simulink model "F1_Simulator"  (R2026a)
settings: Solver=VariableStepAuto  StopTime=260  MaxStep=0.01
values from neighbouring files (symbols this model uses):
  C = [C; C(1,:)]    [f1_corner_map.m]    (also in f1_lateral_tire_table.m = 1.3; f1_sector_map.m = C([true; hypot(diff(C(:,1)), diff(C(:,2))) > 1e-6], :); f1_sensitivity_sweep.m = {; f1_telemetry.m = C([true; hypot(diff(C(:,1)), diff(C(:,2))) > 1e-6], :))
  m = sU >= d0 & sU <= d1    [f1_corner_map.m]    (also in f1_sector_map.m = dC >= edM(k) & dC <= edM(k+1); f1_speed_profile.m = veh.m)
  normalX = -tangentY    [f1_finish_line_params.m]
  normalY = tangentX    [f1_finish_line_params.m]
  s = cumtrapz(tg, v)    [f1_internal_states.m]    (also in f1_track_animation.m = [0; cumsum(hypot(diff(x), diff(y)))]; f1_track_curvature.m = s_all(keepIdx))
  startX = track(1,1)    [f1_finish_line_params.m]
  startY = track(1,2)    [f1_finish_line_params.m]
  tangentX = dirVec(1)    [f1_finish_line_params.m]
  tangentY = dirVec(2)    [f1_finish_line_params.m]
  trackPsi = psi(idx)    [f1_load_raceline.m]    (also in f1_track_curvature.m = atan2(gradient(trackY), gradient(trackX)))
  trackVref = min(trackVref, vf)    [f1_speed_profile.m]
  trackX = x0    [f1_load_raceline.m]    (also in f1_track_curvature.m = x; silverstone_curvature.mat = [-563.032417564 -561.782952087 -560.539483404 -559.300900612)
  trackY = y0    [f1_load_raceline.m]    (also in f1_track_curvature.m = y; silverstone_curvature.mat = [-515.713759288 -514.151171661 -512.584488731 -511.014091481)
undefined symbols (not defined in the file or in its folder): fp_brk_bore, fp_brk_front, fp_brk_maxT, fp_brk_mu_k, fp_brk_pads, fp_brk_Rm, fp_CdA_corner, fp_CdA_straight, fp_eta_tr, fp_gears, fp_h_cg, fp_mu_brake, fp_mu_pk, fp_mu_trac, fp_N_diff, fp_rho, fp_rpm_dn, fp_rpm_lim_end, fp_rpm_lim_ini, fp_rpm_up, fp_track, pwr, veh
libraries: vehdynlibtire x4, autolibsharedcoupling x3, simulink x1, vehdynlibdriver x1, autolibsharedtransfixedgear x1, autolibshareddiff x1, autolibsharedmappedengines x1, autolibshared x1
(part 4 of 5)

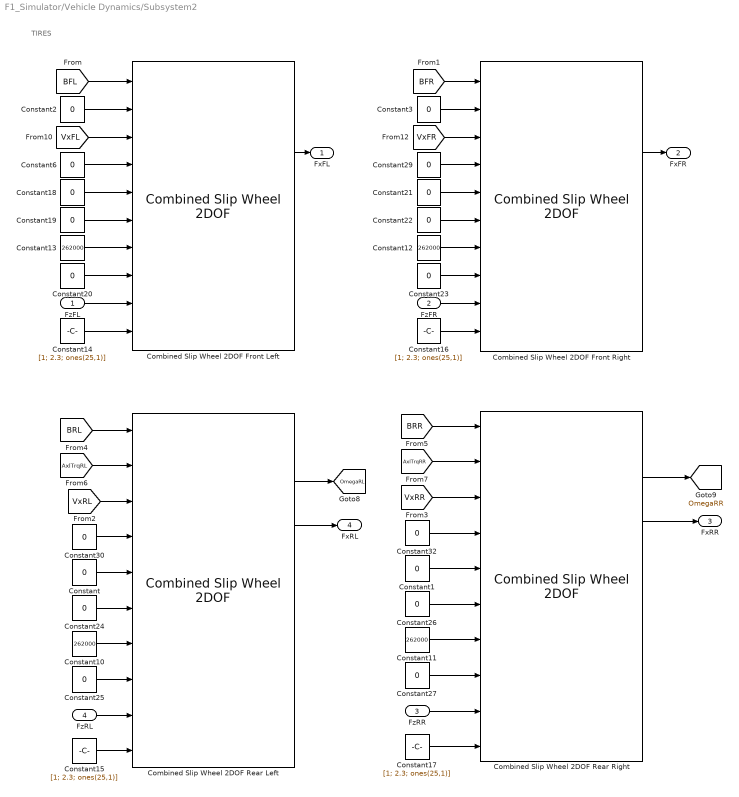
== system F1_Simulator/Vehicle Dynamics/Subsystem2 ==
  note: TIRES
  FzFL : Inport
  FzFR : Inport  Port=2
  FzRR : Inport  Port=3
  FzRL : Inport  Port=4
  Combined Slip Wheel 2DOF Front Left : vehdynlibtire/Combined Slip Wheel 2DOF  tireType=External file  tireParamSet=C:\Users\Julian\Downloads\obfuscated.tir  vertType=Magic Formula  plySteer=on  turnslip=on  BrakeType=Disc  mu_static=0.45  mu_kinetic=brk.mu_k  drum_abore=0.0508  drum_a=0.123  drum_c=0.212  drum_r=0.15  drum_theta1=0  drum_theta2=126  disk_abore=brk.disk_abore  Rm=brk.Rm  num_pads=brk.num_pads  brake_p_bpt=[1 11.4736842105263 21.9473684210526 32.4210526315789 42.8947368421053 53.3684210526316 63.8421052631579 74.3157894736842 84.7894736842105 95.2631578947368 105.736842105263 116.210526315789 126.684210526316 137.157894736842 147.631578947368 158.105263157895 168.578947368421 179.052631578947 189.526315789474 200]  brake_n_bpt=[0 52.6315789473684 105.263157894737 157.894736842105 210.526315789474 263.157894736842 315.789473684211 368.421052631579 421.052631578947 473.684210526316 526.315789473684 578.947368421053 631.578947368421 684.210526315789 736.842105263158 789.473684210526 842.105263157895 894.736842105263 947.368421052632 1000]  f_brake_t=[43.4900602404453 42.5056030554862 41.5350898940194 40.5780454442085 39.6340111501808 38.7025443887544 37.7832176914519 36.8756180088306 35.9793460143796 35.0940154454303 34.2192524787115 33.3546951383474 32.4999927342521 31.6548053290159 30.8188032315107 29.991666515561 29.1730845621415 28.362755623661 27.5603864089927 26.765691687993;498.991217495636 487.695866636631 476.560505099801 465.579679307235 454.748127933653 444.060772460445 433.51270824929 423.099196101319 412.81565427025 402.657650900201 392.620896861006 382.701238955775 372.894653477208 363.197240090814 353.605216024701 344.114910546964 334.722759712992 325.425301366216 316.219170376863 307.10109410434;954.492374750826 932.886130217776 911.585920305583 890.581313170261 869.862244717126 849.419000532136 829.242198807128 809.322774193808 789.651962526121 770.221286354971 751.0225412433 732.047782773203 713.289314220164 694.739674852612 676.391628817892 658.238154578366 640.272434863842 622.48784710877 604.877954344734 587.436496520688;1409.99353200602 1378.07639379892 1346.61133551136 1315.58294703329 1284.9763615006 1254.77722860383 1224.97168936497 1195.5463522863 1166.48827078199 1137.78492180974 1109.42418562559 1081.39432659063 1053.68397496312 1026.28210961441 999.178041611083 972.361398609768 945.822110014692 919.550392851325 893.536738312604 867.771898937035;1865.49468926121 1823.26665738007 1781.63675071715 1740.58458089631 1700.09047828407 1660.13545667552 1620.7011799228 1581.76993037878 1543.32457903786 1505.34855726451 1467.82583000789 1430.74087040806 1394.07863570608 1357.82454437621 1321.96445440427 1286.48464264117 1251.37178516554 1216.61293859388 1182.19552228048 1148.10730135338;2320.9958465164 2268.45692096121 2216.66216592293 2165.58621475934 2115.20459506754 2065.49368474721 2016.43067048064 1967.99350847127 1920.16088729373 1872.91219271928 1826.22747439018 1780.08741422549 1734.47329644903 1689.36697913801 1644.75086719747 1600.60788667257 1556.92146031639 1513.67548433643 1470.85430624835 1428.44270376973;2776.49700377159 2713.64718454235 2651.68758112871 2590.58784862237 2530.31871185102 2470.8519128189 2412.16016103848 2354.21708656376 2296.9971955496 2240.47582817405 2184.62911877248 2129.43395804292 2074.86795719199 2020.9094138998 1967.53727999066 1914.73113070398 1862.47113546724 1810.73803007899 1759.51309021622 1708.77810618608;3231.99816102678 3158.8374481235 3086.71299633449 3015.58948248539 2945.43282863449 2876.21014089059 2807.88965159632 2740.44066465625 2673.83350380547 2608.03946362882 2543.03076315477 2478.78050186034 2415.26261793494 2352.4518486616 2290.32369278385 2228.85437473538 2168.02081061809 2107.80057582154 2048.17187418409 1989.11350860242;3687.49931828197 3604.02771170464 3521.73841154027 3440.59111634842 3360.54694541796 3281.56836896228 3203.61914215416 3126.66424274874 3050.66981206134 2975.60309908359 2901.43240753707 2828.12704567777 2755.6572786779 2683.9942834234 2613.11010557704 2542.97761876678 2473.57048576894 2404.8631215641 2336.83065815196 2269.44891101877;4143.00047553716 4049.21797528579 3956.76382674606 3865.59275021144 3775.66106220143 3686.92659703397 3599.34863271199 3512.88782084123 3427.50612031721 3343.16673453836 3259.83405191936 3177.4735894952 3096.05193942085 3015.5367181852 2935.89651837023 2857.10086279818 2779.12016091979 2701.92566730665 2625.48944211983 2549.78431343512;4598.50163279235 4494.40823886693 4391.78924195184 4290.59438407447 4190.77517898491 4092.28482510566 3995.07812326983 3899.11139893372 3804.34242857308 3710.73036999313 3618.23569630166 3526.82013331263 3436.44660016381 3347.079152947 3258.68293116342 3171.22410682959 3084.66983607064 2998.98821304921 2914.1482260877 2830.11971585147;5054.00279004754 4939.59850244808 4826.81465715762 4715.59601793749 4605.88929576838 4497.64305317735 4390.80761382767 4285.3349770262 4181.17873682896 4078.2940054479 3976.63734068395 3876.16667713006 3776.84126090677 3678.62158770879 3581.46934395661 3485.34735086099 ...(+2764 chars)]  NOMPRES=262000  PRESMAX=1000000  PRESMIN=10000  FNOMIN=tire.Fz0_roll  FZMAX=tire.FZMAX  FZMIN=100  VXLOW=1  KPUMAX=1.5  KPUMIN=-1.5  ALPMAX=1.5  ALPMIN=-1.5  CAMMAX=0.17453  CAMMIN=-0.17453  LONGVL=16.7  FxRelFreqLwrLim=40*pi  FyRelFreqLwrLim=0  MyRelFreqLwrLim=40*pi  omegao=0  UNLOADED_RADIUS=0.353  WIDTH=0.280  RIM_RADIUS=0.2286  ASPECT_RATIO=0.45  MASS=11.2  IYY=1.084  br=0.01  GRAVITY=-9.81  zo=0  zdoto=0  BREFF=8.25094594147963  DREFF=0.260468730454265  FREFF=0.0735298544471851  Q_RE0=1.00866439868088  Q_V1=0.000760413786224011  Q_V2=0.0463384792019201  Q_FZ1=0  Q_FZ2=15.6870832810226  Q_FZ3=0  Q_FCX=0.138643970247602  Q_FCY=0.10843499565426  Q_FCY2=-0.465763352339538  PFZ1=0.69958166705601  VERTICAL_STIFFNESS=207885.061134007  VERTICAL_DAMPING=500  BOTTOM_OFFST=0.00990653336182505  BOTTOM_STIFF=1999075.87051971  Q_CAM1=86.7791723017291  Q_CAM2=259.705254231766  Q_CAM3=0.510281667378416  Q_FYS1=-20769.4728880343  Q_FYS2=-59060.183485617  Q_FYS3=89271.8260126986  LONGITUDINAL_STIFFNESS=388714.175879854  LATERAL_STIFFNESS=157087.404633332  PCFX1=0.18539229191199  PCFX2=0  PCFX3=0  PCFY1=0.163183345037677  PCFY2=0  PCFY3=0.249094918231954  Q_RA1=0.675942571700787  Q_RA2=0.73800463546164  Q_RB1=1.04487486456705  Q_RB2=-1.191763806629  PCX1=1.58523057950359  PDX1=1.7  PDX2=-0.0842405110022724  PDX3=0  PEX1=0.110312777158455  PEX2=0.313468516038146  PEX3=0  PEX4=0.0016060905760045  PKX1=21.3872544684023  PKX2=14.0006541873175  PKX3=-0.405326109653452  PHX1=0.000212599305364818  PHX2=0.00115950515263055  PVX1=1.59236164471432e-05  PVX2=0.000104321112127671  PPX1=-0.349461321276586  PPX2=0.387840040616429  PPX3=-0.0969947336569324  PPX4=0.0632271859795801  RBX1=12.7633329850276  RBX2=9.5787123658471  RBX3=0  RCX1=1.02796280922059  REX1=-0.45202516851367  REX2=-0.47304886171176  RHX1=0.000233272373115809  QSX1=-0.00788307788961443  QSX2=0.954629515459396  QSX3=0.0155855777667025  QSX4=0.125904607142414  QSX5=1.01110069703963  QSX6=20.1938577118433  QSX7=0.310818120717083  QSX8=-0.0430823751139655  QSX9=0.636494404888216  QSX10=0.142438060591663  QSX11=0.346766530036373  QSX12=0  QSX13=0  QSX14=0  PPMX1=0  PCY1=1.34299950037631  PDY1=0.878267729082195  PDY2=-0.0644597923147385  PDY3=0  PEY1=-0.809776534470972  PEY2=-0.600180598867198  PEY3=0.0991732552633487  PEY4=-6.5577974035573  PEY5=0  PKY1=-15.5714726518315  PKY2=1.73126522291751  PKY3=0.365349873517229  PKY4=1.98176755955416  PKY5=0  PKY6=-0.884005199550313  PKY7=-0.237259727611847  PHY1=-0.00183370557235628  PHY2=0.00346401302716671  PVY1=-0.00675427560163264  PVY2=0.036379218103843  PVY3=-0.163543984089166  PVY4=-0.491003349625726  PPY1=-0.62059646553185  PPY2=-0.0647824842338686  PPY3=-0.164648843290686  PPY4=0.283193909060098  PPY5=0  RBY1=10.7588809173639  RBY2=7.70420065295029  RBY3=3.40283755070691e-06  RBY4=0  RCY1=1.06691874059059  REY1=0.308244924574305  REY2=7.48775032604508e-06  RHY1=0.0118479204960415  RHY2=7.63650177161071e-06  RVY1=0.0560024425050078  RVY2=7.48487127056197e-06  RVY3=0  RVY4=98.4047026517149  RVY5=2.02759273900054  RVY6=15.7623064923347  QSY1=0.00699077564863536  QSY2=0  QSY3=0.00153535478298811  QSY4=8.55710322455322e-05  QSY5=0  QSY6=0  QSY7=0.89443879773793  QSY8=-0.403227641260894  QBZ1=11.666656027484  QBZ2=-1.30355438574485  QBZ3=0  QBZ4=0.177918305399071  QBZ5=-0.162481135068033  QBZ6=0  QBZ9=30.1445534682089  QBZ10=0  QCZ1=1.29026978207574  QDZ1=0.0886972644991399  QDZ2=-0.0058634820161856  QDZ3=0.3805597481383  QDZ4=0  QDZ6=0.00160914918118959  QDZ7=-0.00211036330862154  QDZ8=-0.13921904912557  QDZ9=0.00816585550028243  QDZ10=0  QDZ11=0  QEZ1=-2.19802254534746  QEZ2=1.01850535789165  QEZ3=0  QEZ4=0.278379679112054  QEZ5=-0.548414722765386  QHZ1=0.00148361198869669  QHZ2=0.00202017567585904  QHZ3=0.240316641332066  QHZ4=-0.210114035738085  PPZ1=-0.443927982388615  PPZ2=0  SSZ1=0.00914999585397887  SSZ2=0.0389830656052735  SSZ3=0  SSZ4=0  PDXP1=0.396718274678791  PDXP2=0  PDXP3=0  PKYP1=1.00587060633573  PDYP1=0.40483048923438  PDYP2=0  PDYP3=0  PDYP4=0  PHYP1=0.992731942067188  PHYP2=0.150352945499914  PHYP3=0  PHYP4=-3.98988682633674  PECP1=0.502379254513503  PECP2=0  QDTP1=10.0178654287947  QCRP1=0.200627747200702  QCRP2=0.0995735881599772  QBRP1=0.0997107127960717  QDRP1=1.01432910167423  QDRP2=0  aMode=2
  Combined Slip Wheel 2DOF Front Right : vehdynlibtire/Combined Slip Wheel 2DOF  tireType=External file  tireParamSet=C:\Users\Julian\Downloads\obfuscated.tir  vertType=Magic Formula  plySteer=on  turnslip=on  BrakeType=Disc  mu_static=0.45  mu_kinetic=brk.mu_k  drum_abore=0.0508  drum_a=0.123  drum_c=0.212  drum_r=0.15  drum_theta1=0  drum_theta2=126  disk_abore=brk.disk_abore  Rm=brk.Rm  num_pads=brk.num_pads  brake_p_bpt=[1 11.4736842105263 21.9473684210526 32.4210526315789 42.8947368421053 53.3684210526316 63.8421052631579 74.3157894736842 84.7894736842105 95.2631578947368 105.736842105263 116.210526315789 126.684210526316 137.157894736842 147.631578947368 158.105263157895 168.578947368421 179.052631578947 189.526315789474 200]  brake_n_bpt=[0 52.6315789473684 105.263157894737 157.894736842105 210.526315789474 263.157894736842 315.789473684211 368.421052631579 421.052631578947 473.684210526316 526.315789473684 578.947368421053 631.578947368421 684.210526315789 736.842105263158 789.473684210526 842.105263157895 894.736842105263 947.368421052632 1000]  f_brake_t=[43.4900602404453 42.5056030554862 41.5350898940194 40.5780454442085 39.6340111501808 38.7025443887544 37.7832176914519 36.8756180088306 35.9793460143796 35.0940154454303 34.2192524787115 33.3546951383474 32.4999927342521 31.6548053290159 30.8188032315107 29.991666515561 29.1730845621415 28.362755623661 27.5603864089927 26.765691687993;498.991217495636 487.695866636631 476.560505099801 465.579679307235 454.748127933653 444.060772460445 433.51270824929 423.099196101319 412.81565427025 402.657650900201 392.620896861006 382.701238955775 372.894653477208 363.197240090814 353.605216024701 344.114910546964 334.722759712992 325.425301366216 316.219170376863 307.10109410434;954.492374750826 932.886130217776 911.585920305583 890.581313170261 869.862244717126 849.419000532136 829.242198807128 809.322774193808 789.651962526121 770.221286354971 751.0225412433 732.047782773203 713.289314220164 694.739674852612 676.391628817892 658.238154578366 640.272434863842 622.48784710877 604.877954344734 587.436496520688;1409.99353200602 1378.07639379892 1346.61133551136 1315.58294703329 1284.9763615006 1254.77722860383 1224.97168936497 1195.5463522863 1166.48827078199 1137.78492180974 1109.42418562559 1081.39432659063 1053.68397496312 1026.28210961441 999.178041611083 972.361398609768 945.822110014692 919.550392851325 893.536738312604 867.771898937035;1865.49468926121 1823.26665738007 1781.63675071715 1740.58458089631 1700.09047828407 1660.13545667552 1620.7011799228 1581.76993037878 1543.32457903786 1505.34855726451 1467.82583000789 1430.74087040806 1394.07863570608 1357.82454437621 1321.96445440427 1286.48464264117 1251.37178516554 1216.61293859388 1182.19552228048 1148.10730135338;2320.9958465164 2268.45692096121 2216.66216592293 2165.58621475934 2115.20459506754 2065.49368474721 2016.43067048064 1967.99350847127 1920.16088729373 1872.91219271928 1826.22747439018 1780.08741422549 1734.47329644903 1689.36697913801 1644.75086719747 1600.60788667257 1556.92146031639 1513.67548433643 1470.85430624835 1428.44270376973;2776.49700377159 2713.64718454235 2651.68758112871 2590.58784862237 2530.31871185102 2470.8519128189 2412.16016103848 2354.21708656376 2296.9971955496 2240.47582817405 2184.62911877248 2129.43395804292 2074.86795719199 2020.9094138998 1967.53727999066 1914.73113070398 1862.47113546724 1810.73803007899 1759.51309021622 1708.77810618608;3231.99816102678 3158.8374481235 3086.71299633449 3015.58948248539 2945.43282863449 2876.21014089059 2807.88965159632 2740.44066465625 2673.83350380547 2608.03946362882 2543.03076315477 2478.78050186034 2415.26261793494 2352.4518486616 2290.32369278385 2228.85437473538 2168.02081061809 2107.80057582154 2048.17187418409 1989.11350860242;3687.49931828197 3604.02771170464 3521.73841154027 3440.59111634842 3360.54694541796 3281.56836896228 3203.61914215416 3126.66424274874 3050.66981206134 2975.60309908359 2901.43240753707 2828.12704567777 2755.6572786779 2683.9942834234 2613.11010557704 2542.97761876678 2473.57048576894 2404.8631215641 2336.83065815196 2269.44891101877;4143.00047553716 4049.21797528579 3956.76382674606 3865.59275021144 3775.66106220143 3686.92659703397 3599.34863271199 3512.88782084123 3427.50612031721 3343.16673453836 3259.83405191936 3177.4735894952 3096.05193942085 3015.5367181852 2935.89651837023 2857.10086279818 2779.12016091979 2701.92566730665 2625.48944211983 2549.78431343512;4598.50163279235 4494.40823886693 4391.78924195184 4290.59438407447 4190.77517898491 4092.28482510566 3995.07812326983 3899.11139893372 3804.34242857308 3710.73036999313 3618.23569630166 3526.82013331263 3436.44660016381 3347.079152947 3258.68293116342 3171.22410682959 3084.66983607064 2998.98821304921 2914.1482260877 2830.11971585147;5054.00279004754 4939.59850244808 4826.81465715762 4715.59601793749 4605.88929576838 4497.64305317735 4390.80761382767 4285.3349770262 4181.17873682896 4078.2940054479 3976.63734068395 3876.16667713006 3776.84126090677 3678.62158770879 3581.46934395661 3485.34735086099 ...(+2764 chars)]  NOMPRES=262000  PRESMAX=1000000  PRESMIN=10000  FNOMIN=tire.Fz0_roll  FZMAX=tire.FZMAX  FZMIN=100  VXLOW=1  KPUMAX=1.5  KPUMIN=-1.5  ALPMAX=1.5  ALPMIN=-1.5  CAMMAX=0.17453  CAMMIN=-0.17453  LONGVL=16.7  FxRelFreqLwrLim=40*pi  FyRelFreqLwrLim=0  MyRelFreqLwrLim=40*pi  omegao=0  UNLOADED_RADIUS=0.353  WIDTH=0.280  RIM_RADIUS=0.2286  ASPECT_RATIO=0.45  MASS=11.2  IYY=1.084  br=0.01  GRAVITY=-9.81  zo=0  zdoto=0  BREFF=8.25094594147963  DREFF=0.260468730454265  FREFF=0.0735298544471851  Q_RE0=1.00866439868088  Q_V1=0.000760413786224011  Q_V2=0.0463384792019201  Q_FZ1=0  Q_FZ2=15.6870832810226  Q_FZ3=0  Q_FCX=0.138643970247602  Q_FCY=0.10843499565426  Q_FCY2=-0.465763352339538  PFZ1=0.69958166705601  VERTICAL_STIFFNESS=207885.061134007  VERTICAL_DAMPING=500  BOTTOM_OFFST=0.00990653336182505  BOTTOM_STIFF=1999075.87051971  Q_CAM1=86.7791723017291  Q_CAM2=259.705254231766  Q_CAM3=0.510281667378416  Q_FYS1=-20769.4728880343  Q_FYS2=-59060.183485617  Q_FYS3=89271.8260126986  LONGITUDINAL_STIFFNESS=388714.175879854  LATERAL_STIFFNESS=157087.404633332  PCFX1=0.18539229191199  PCFX2=0  PCFX3=0  PCFY1=0.163183345037677  PCFY2=0  PCFY3=0.249094918231954  Q_RA1=0.675942571700787  Q_RA2=0.73800463546164  Q_RB1=1.04487486456705  Q_RB2=-1.191763806629  PCX1=1.58523057950359  PDX1=1.7  PDX2=-0.0842405110022724  PDX3=0  PEX1=0.110312777158455  PEX2=0.313468516038146  PEX3=0  PEX4=0.0016060905760045  PKX1=21.3872544684023  PKX2=14.0006541873175  PKX3=-0.405326109653452  PHX1=0.000212599305364818  PHX2=0.00115950515263055  PVX1=1.59236164471432e-05  PVX2=0.000104321112127671  PPX1=-0.349461321276586  PPX2=0.387840040616429  PPX3=-0.0969947336569324  PPX4=0.0632271859795801  RBX1=12.7633329850276  RBX2=9.5787123658471  RBX3=0  RCX1=1.02796280922059  REX1=-0.45202516851367  REX2=-0.47304886171176  RHX1=0.000233272373115809  QSX1=-0.00788307788961443  QSX2=0.954629515459396  QSX3=0.0155855777667025  QSX4=0.125904607142414  QSX5=1.01110069703963  QSX6=20.1938577118433  QSX7=0.310818120717083  QSX8=-0.0430823751139655  QSX9=0.636494404888216  QSX10=0.142438060591663  QSX11=0.346766530036373  QSX12=0  QSX13=0  QSX14=0  PPMX1=0  PCY1=1.34299950037631  PDY1=0.878267729082195  PDY2=-0.0644597923147385  PDY3=0  PEY1=-0.809776534470972  PEY2=-0.600180598867198  PEY3=0.0991732552633487  PEY4=-6.5577974035573  PEY5=0  PKY1=-15.5714726518315  PKY2=1.73126522291751  PKY3=0.365349873517229  PKY4=1.98176755955416  PKY5=0  PKY6=-0.884005199550313  PKY7=-0.237259727611847  PHY1=-0.00183370557235628  PHY2=0.00346401302716671  PVY1=-0.00675427560163264  PVY2=0.036379218103843  PVY3=-0.163543984089166  PVY4=-0.491003349625726  PPY1=-0.62059646553185  PPY2=-0.0647824842338686  PPY3=-0.164648843290686  PPY4=0.283193909060098  PPY5=0  RBY1=10.7588809173639  RBY2=7.70420065295029  RBY3=3.40283755070691e-06  RBY4=0  RCY1=1.06691874059059  REY1=0.308244924574305  REY2=7.48775032604508e-06  RHY1=0.0118479204960415  RHY2=7.63650177161071e-06  RVY1=0.0560024425050078  RVY2=7.48487127056197e-06  RVY3=0  RVY4=98.4047026517149  RVY5=2.02759273900054  RVY6=15.7623064923347  QSY1=0.00699077564863536  QSY2=0  QSY3=0.00153535478298811  QSY4=8.55710322455322e-05  QSY5=0  QSY6=0  QSY7=0.89443879773793  QSY8=-0.403227641260894  QBZ1=11.666656027484  QBZ2=-1.30355438574485  QBZ3=0  QBZ4=0.177918305399071  QBZ5=-0.162481135068033  QBZ6=0  QBZ9=30.1445534682089  QBZ10=0  QCZ1=1.29026978207574  QDZ1=0.0886972644991399  QDZ2=-0.0058634820161856  QDZ3=0.3805597481383  QDZ4=0  QDZ6=0.00160914918118959  QDZ7=-0.00211036330862154  QDZ8=-0.13921904912557  QDZ9=0.00816585550028243  QDZ10=0  QDZ11=0  QEZ1=-2.19802254534746  QEZ2=1.01850535789165  QEZ3=0  QEZ4=0.278379679112054  QEZ5=-0.548414722765386  QHZ1=0.00148361198869669  QHZ2=0.00202017567585904  QHZ3=0.240316641332066  QHZ4=-0.210114035738085  PPZ1=-0.443927982388615  PPZ2=0  SSZ1=0.00914999585397887  SSZ2=0.0389830656052735  SSZ3=0  SSZ4=0  PDXP1=0.396718274678791  PDXP2=0  PDXP3=0  PKYP1=1.00587060633573  PDYP1=0.40483048923438  PDYP2=0  PDYP3=0  PDYP4=0  PHYP1=0.992731942067188  PHYP2=0.150352945499914  PHYP3=0  PHYP4=-3.98988682633674  PECP1=0.502379254513503  PECP2=0  QDTP1=10.0178654287947  QCRP1=0.200627747200702  QCRP2=0.0995735881599772  QBRP1=0.0997107127960717  QDRP1=1.01432910167423  QDRP2=0  aMode=2
  Combined Slip Wheel 2DOF Rear Left : vehdynlibtire/Combined Slip Wheel 2DOF  tireType=External file  tireParamSet=C:\Users\Julian\Downloads\obfuscated.tir  vertType=Magic Formula  plySteer=on  turnslip=on  BrakeType=Disc  mu_static=0.45  mu_kinetic=brk.mu_k  drum_abore=0.0508  drum_a=0.123  drum_c=0.212  drum_r=0.15  drum_theta1=0  drum_theta2=126  disk_abore=brk.disk_abore  Rm=brk.Rm  num_pads=brk.num_pads  brake_p_bpt=[1 11.4736842105263 21.9473684210526 32.4210526315789 42.8947368421053 53.3684210526316 63.8421052631579 74.3157894736842 84.7894736842105 95.2631578947368 105.736842105263 116.210526315789 126.684210526316 137.157894736842 147.631578947368 158.105263157895 168.578947368421 179.052631578947 189.526315789474 200]  brake_n_bpt=[0 52.6315789473684 105.263157894737 157.894736842105 210.526315789474 263.157894736842 315.789473684211 368.421052631579 421.052631578947 473.684210526316 526.315789473684 578.947368421053 631.578947368421 684.210526315789 736.842105263158 789.473684210526 842.105263157895 894.736842105263 947.368421052632 1000]  f_brake_t=[43.4900602404453 42.5056030554862 41.5350898940194 40.5780454442085 39.6340111501808 38.7025443887544 37.7832176914519 36.8756180088306 35.9793460143796 35.0940154454303 34.2192524787115 33.3546951383474 32.4999927342521 31.6548053290159 30.8188032315107 29.991666515561 29.1730845621415 28.362755623661 27.5603864089927 26.765691687993;498.991217495636 487.695866636631 476.560505099801 465.579679307235 454.748127933653 444.060772460445 433.51270824929 423.099196101319 412.81565427025 402.657650900201 392.620896861006 382.701238955775 372.894653477208 363.197240090814 353.605216024701 344.114910546964 334.722759712992 325.425301366216 316.219170376863 307.10109410434;954.492374750826 932.886130217776 911.585920305583 890.581313170261 869.862244717126 849.419000532136 829.242198807128 809.322774193808 789.651962526121 770.221286354971 751.0225412433 732.047782773203 713.289314220164 694.739674852612 676.391628817892 658.238154578366 640.272434863842 622.48784710877 604.877954344734 587.436496520688;1409.99353200602 1378.07639379892 1346.61133551136 1315.58294703329 1284.9763615006 1254.77722860383 1224.97168936497 1195.5463522863 1166.48827078199 1137.78492180974 1109.42418562559 1081.39432659063 1053.68397496312 1026.28210961441 999.178041611083 972.361398609768 945.822110014692 919.550392851325 893.536738312604 867.771898937035;1865.49468926121 1823.26665738007 1781.63675071715 1740.58458089631 1700.09047828407 1660.13545667552 1620.7011799228 1581.76993037878 1543.32457903786 1505.34855726451 1467.82583000789 1430.74087040806 1394.07863570608 1357.82454437621 1321.96445440427 1286.48464264117 1251.37178516554 1216.61293859388 1182.19552228048 1148.10730135338;2320.9958465164 2268.45692096121 2216.66216592293 2165.58621475934 2115.20459506754 2065.49368474721 2016.43067048064 1967.99350847127 1920.16088729373 1872.91219271928 1826.22747439018 1780.08741422549 1734.47329644903 1689.36697913801 1644.75086719747 1600.60788667257 1556.92146031639 1513.67548433643 1470.85430624835 1428.44270376973;2776.49700377159 2713.64718454235 2651.68758112871 2590.58784862237 2530.31871185102 2470.8519128189 2412.16016103848 2354.21708656376 2296.9971955496 2240.47582817405 2184.62911877248 2129.43395804292 2074.86795719199 2020.9094138998 1967.53727999066 1914.73113070398 1862.47113546724 1810.73803007899 1759.51309021622 1708.77810618608;3231.99816102678 3158.8374481235 3086.71299633449 3015.58948248539 2945.43282863449 2876.21014089059 2807.88965159632 2740.44066465625 2673.83350380547 2608.03946362882 2543.03076315477 2478.78050186034 2415.26261793494 2352.4518486616 2290.32369278385 2228.85437473538 2168.02081061809 2107.80057582154 2048.17187418409 1989.11350860242;3687.49931828197 3604.02771170464 3521.73841154027 3440.59111634842 3360.54694541796 3281.56836896228 3203.61914215416 3126.66424274874 3050.66981206134 2975.60309908359 2901.43240753707 2828.12704567777 2755.6572786779 2683.9942834234 2613.11010557704 2542.97761876678 2473.57048576894 2404.8631215641 2336.83065815196 2269.44891101877;4143.00047553716 4049.21797528579 3956.76382674606 3865.59275021144 3775.66106220143 3686.92659703397 3599.34863271199 3512.88782084123 3427.50612031721 3343.16673453836 3259.83405191936 3177.4735894952 3096.05193942085 3015.5367181852 2935.89651837023 2857.10086279818 2779.12016091979 2701.92566730665 2625.48944211983 2549.78431343512;4598.50163279235 4494.40823886693 4391.78924195184 4290.59438407447 4190.77517898491 4092.28482510566 3995.07812326983 3899.11139893372 3804.34242857308 3710.73036999313 3618.23569630166 3526.82013331263 3436.44660016381 3347.079152947 3258.68293116342 3171.22410682959 3084.66983607064 2998.98821304921 2914.1482260877 2830.11971585147;5054.00279004754 4939.59850244808 4826.81465715762 4715.59601793749 4605.88929576838 4497.64305317735 4390.80761382767 4285.3349770262 4181.17873682896 4078.2940054479 3976.63734068395 3876.16667713006 3776.84126090677 3678.62158770879 3581.46934395661 3485.34735086099 ...(+2764 chars)]  NOMPRES=262000  PRESMAX=1000000  PRESMIN=10000  FNOMIN=tire.Fz0_roll  FZMAX=tire.FZMAX  FZMIN=100  VXLOW=1  KPUMAX=1.5  KPUMIN=-1.5  ALPMAX=1.5  ALPMIN=-1.5  CAMMAX=0.17453  CAMMIN=-0.17453  LONGVL=16.7  FxRelFreqLwrLim=40*pi  FyRelFreqLwrLim=0  MyRelFreqLwrLim=40*pi  omegao=0  UNLOADED_RADIUS=0.353  WIDTH=0.375  RIM_RADIUS=0.2286  ASPECT_RATIO=0.45  MASS=11.2  IYY=1.084  br=0.01  GRAVITY=-9.81  zo=0  zdoto=0  BREFF=8.25094594147963  DREFF=0.260468730454265  FREFF=0.0735298544471851  Q_RE0=1.00866439868088  Q_V1=0.000760413786224011  Q_V2=0.0463384792019201  Q_FZ1=0  Q_FZ2=15.6870832810226  Q_FZ3=0  Q_FCX=0.138643970247602  Q_FCY=0.10843499565426  Q_FCY2=-0.465763352339538  PFZ1=0.69958166705601  VERTICAL_STIFFNESS=207885.061134007  VERTICAL_DAMPING=500  BOTTOM_OFFST=0.00990653336182505  BOTTOM_STIFF=1999075.87051971  Q_CAM1=86.7791723017291  Q_CAM2=259.705254231766  Q_CAM3=0.510281667378416  Q_FYS1=-20769.4728880343  Q_FYS2=-59060.183485617  Q_FYS3=89271.8260126986  LONGITUDINAL_STIFFNESS=388714.175879854  LATERAL_STIFFNESS=157087.404633332  PCFX1=0.18539229191199  PCFX2=0  PCFX3=0  PCFY1=0.163183345037677  PCFY2=0  PCFY3=0.249094918231954  Q_RA1=0.675942571700787  Q_RA2=0.73800463546164  Q_RB1=1.04487486456705  Q_RB2=-1.191763806629  PCX1=1.58523057950359  PDX1=1.7  PDX2=-0.0842405110022724  PDX3=0  PEX1=0.110312777158455  PEX2=0.313468516038146  PEX3=0  PEX4=0.0016060905760045  PKX1=21.3872544684023  PKX2=14.0006541873175  PKX3=-0.405326109653452  PHX1=0.000212599305364818  PHX2=0.00115950515263055  PVX1=1.59236164471432e-05  PVX2=0.000104321112127671  PPX1=-0.349461321276586  PPX2=0.387840040616429  PPX3=-0.0969947336569324  PPX4=0.0632271859795801  RBX1=12.7633329850276  RBX2=9.5787123658471  RBX3=0  RCX1=1.02796280922059  REX1=-0.45202516851367  REX2=-0.47304886171176  RHX1=0.000233272373115809  QSX1=-0.00788307788961443  QSX2=0.954629515459396  QSX3=0.0155855777667025  QSX4=0.125904607142414  QSX5=1.01110069703963  QSX6=20.1938577118433  QSX7=0.310818120717083  QSX8=-0.0430823751139655  QSX9=0.636494404888216  QSX10=0.142438060591663  QSX11=0.346766530036373  QSX12=0  QSX13=0  QSX14=0  PPMX1=0  PCY1=1.34299950037631  PDY1=0.878267729082195  PDY2=-0.0644597923147385  PDY3=0  PEY1=-0.809776534470972  PEY2=-0.600180598867198  PEY3=0.0991732552633487  PEY4=-6.5577974035573  PEY5=0  PKY1=-15.5714726518315  PKY2=1.73126522291751  PKY3=0.365349873517229  PKY4=1.98176755955416  PKY5=0  PKY6=-0.884005199550313  PKY7=-0.237259727611847  PHY1=-0.00183370557235628  PHY2=0.00346401302716671  PVY1=-0.00675427560163264  PVY2=0.036379218103843  PVY3=-0.163543984089166  PVY4=-0.491003349625726  PPY1=-0.62059646553185  PPY2=-0.0647824842338686  PPY3=-0.164648843290686  PPY4=0.283193909060098  PPY5=0  RBY1=10.7588809173639  RBY2=7.70420065295029  RBY3=3.40283755070691e-06  RBY4=0  RCY1=1.06691874059059  REY1=0.308244924574305  REY2=7.48775032604508e-06  RHY1=0.0118479204960415  RHY2=7.63650177161071e-06  RVY1=0.0560024425050078  RVY2=7.48487127056197e-06  RVY3=0  RVY4=98.4047026517149  RVY5=2.02759273900054  RVY6=15.7623064923347  QSY1=0.00699077564863536  QSY2=0  QSY3=0.00153535478298811  QSY4=8.55710322455322e-05  QSY5=0  QSY6=0  QSY7=0.89443879773793  QSY8=-0.403227641260894  QBZ1=11.666656027484  QBZ2=-1.30355438574485  QBZ3=0  QBZ4=0.177918305399071  QBZ5=-0.162481135068033  QBZ6=0  QBZ9=30.1445534682089  QBZ10=0  QCZ1=1.29026978207574  QDZ1=0.0886972644991399  QDZ2=-0.0058634820161856  QDZ3=0.3805597481383  QDZ4=0  QDZ6=0.00160914918118959  QDZ7=-0.00211036330862154  QDZ8=-0.13921904912557  QDZ9=0.00816585550028243  QDZ10=0  QDZ11=0  QEZ1=-2.19802254534746  QEZ2=1.01850535789165  QEZ3=0  QEZ4=0.278379679112054  QEZ5=-0.548414722765386  QHZ1=0.00148361198869669  QHZ2=0.00202017567585904  QHZ3=0.240316641332066  QHZ4=-0.210114035738085  PPZ1=-0.443927982388615  PPZ2=0  SSZ1=0.00914999585397887  SSZ2=0.0389830656052735  SSZ3=0  SSZ4=0  PDXP1=0.396718274678791  PDXP2=0  PDXP3=0  PKYP1=1.00587060633573  PDYP1=0.40483048923438  PDYP2=0  PDYP3=0  PDYP4=0  PHYP1=0.992731942067188  PHYP2=0.150352945499914  PHYP3=0  PHYP4=-3.98988682633674  PECP1=0.502379254513503  PECP2=0  QDTP1=10.0178654287947  QCRP1=0.200627747200702  QCRP2=0.0995735881599772  QBRP1=0.0997107127960717  QDRP1=1.01432910167423  QDRP2=0  aMode=2
  Combined Slip Wheel 2DOF Rear Right : vehdynlibtire/Combined Slip Wheel 2DOF  tireType=External file  tireParamSet=C:\Users\Julian\Downloads\obfuscated.tir  vertType=Magic Formula  plySteer=on  turnslip=on  BrakeType=Disc  mu_static=0.45  mu_kinetic=brk.mu_k  drum_abore=0.0508  drum_a=0.123  drum_c=0.212  drum_r=0.15  drum_theta1=0  drum_theta2=126  disk_abore=brk.disk_abore  Rm=brk.Rm  num_pads=brk.num_pads  brake_p_bpt=[1 11.4736842105263 21.9473684210526 32.4210526315789 42.8947368421053 53.3684210526316 63.8421052631579 74.3157894736842 84.7894736842105 95.2631578947368 105.736842105263 116.210526315789 126.684210526316 137.157894736842 147.631578947368 158.105263157895 168.578947368421 179.052631578947 189.526315789474 200]  brake_n_bpt=[0 52.6315789473684 105.263157894737 157.894736842105 210.526315789474 263.157894736842 315.789473684211 368.421052631579 421.052631578947 473.684210526316 526.315789473684 578.947368421053 631.578947368421 684.210526315789 736.842105263158 789.473684210526 842.105263157895 894.736842105263 947.368421052632 1000]  f_brake_t=[43.4900602404453 42.5056030554862 41.5350898940194 40.5780454442085 39.6340111501808 38.7025443887544 37.7832176914519 36.8756180088306 35.9793460143796 35.0940154454303 34.2192524787115 33.3546951383474 32.4999927342521 31.6548053290159 30.8188032315107 29.991666515561 29.1730845621415 28.362755623661 27.5603864089927 26.765691687993;498.991217495636 487.695866636631 476.560505099801 465.579679307235 454.748127933653 444.060772460445 433.51270824929 423.099196101319 412.81565427025 402.657650900201 392.620896861006 382.701238955775 372.894653477208 363.197240090814 353.605216024701 344.114910546964 334.722759712992 325.425301366216 316.219170376863 307.10109410434;954.492374750826 932.886130217776 911.585920305583 890.581313170261 869.862244717126 849.419000532136 829.242198807128 809.322774193808 789.651962526121 770.221286354971 751.0225412433 732.047782773203 713.289314220164 694.739674852612 676.391628817892 658.238154578366 640.272434863842 622.48784710877 604.877954344734 587.436496520688;1409.99353200602 1378.07639379892 1346.61133551136 1315.58294703329 1284.9763615006 1254.77722860383 1224.97168936497 1195.5463522863 1166.48827078199 1137.78492180974 1109.42418562559 1081.39432659063 1053.68397496312 1026.28210961441 999.178041611083 972.361398609768 945.822110014692 919.550392851325 893.536738312604 867.771898937035;1865.49468926121 1823.26665738007 1781.63675071715 1740.58458089631 1700.09047828407 1660.13545667552 1620.7011799228 1581.76993037878 1543.32457903786 1505.34855726451 1467.82583000789 1430.74087040806 1394.07863570608 1357.82454437621 1321.96445440427 1286.48464264117 1251.37178516554 1216.61293859388 1182.19552228048 1148.10730135338;2320.9958465164 2268.45692096121 2216.66216592293 2165.58621475934 2115.20459506754 2065.49368474721 2016.43067048064 1967.99350847127 1920.16088729373 1872.91219271928 1826.22747439018 1780.08741422549 1734.47329644903 1689.36697913801 1644.75086719747 1600.60788667257 1556.92146031639 1513.67548433643 1470.85430624835 1428.44270376973;2776.49700377159 2713.64718454235 2651.68758112871 2590.58784862237 2530.31871185102 2470.8519128189 2412.16016103848 2354.21708656376 2296.9971955496 2240.47582817405 2184.62911877248 2129.43395804292 2074.86795719199 2020.9094138998 1967.53727999066 1914.73113070398 1862.47113546724 1810.73803007899 1759.51309021622 1708.77810618608;3231.99816102678 3158.8374481235 3086.71299633449 3015.58948248539 2945.43282863449 2876.21014089059 2807.88965159632 2740.44066465625 2673.83350380547 2608.03946362882 2543.03076315477 2478.78050186034 2415.26261793494 2352.4518486616 2290.32369278385 2228.85437473538 2168.02081061809 2107.80057582154 2048.17187418409 1989.11350860242;3687.49931828197 3604.02771170464 3521.73841154027 3440.59111634842 3360.54694541796 3281.56836896228 3203.61914215416 3126.66424274874 3050.66981206134 2975.60309908359 2901.43240753707 2828.12704567777 2755.6572786779 2683.9942834234 2613.11010557704 2542.97761876678 2473.57048576894 2404.8631215641 2336.83065815196 2269.44891101877;4143.00047553716 4049.21797528579 3956.76382674606 3865.59275021144 3775.66106220143 3686.92659703397 3599.34863271199 3512.88782084123 3427.50612031721 3343.16673453836 3259.83405191936 3177.4735894952 3096.05193942085 3015.5367181852 2935.89651837023 2857.10086279818 2779.12016091979 2701.92566730665 2625.48944211983 2549.78431343512;4598.50163279235 4494.40823886693 4391.78924195184 4290.59438407447 4190.77517898491 4092.28482510566 3995.07812326983 3899.11139893372 3804.34242857308 3710.73036999313 3618.23569630166 3526.82013331263 3436.44660016381 3347.079152947 3258.68293116342 3171.22410682959 3084.66983607064 2998.98821304921 2914.1482260877 2830.11971585147;5054.00279004754 4939.59850244808 4826.81465715762 4715.59601793749 4605.88929576838 4497.64305317735 4390.80761382767 4285.3349770262 4181.17873682896 4078.2940054479 3976.63734068395 3876.16667713006 3776.84126090677 3678.62158770879 3581.46934395661 3485.34735086099 ...(+2764 chars)]  NOMPRES=262000  PRESMAX=1000000  PRESMIN=10000  FNOMIN=tire.Fz0_roll  FZMAX=tire.FZMAX  FZMIN=100  VXLOW=1  KPUMAX=1.5  KPUMIN=-1.5  ALPMAX=1.5  ALPMIN=-1.5  CAMMAX=0.17453  CAMMIN=-0.17453  LONGVL=16.7  FxRelFreqLwrLim=40*pi  FyRelFreqLwrLim=0  MyRelFreqLwrLim=40*pi  omegao=0  UNLOADED_RADIUS=0.353  WIDTH=0.375  RIM_RADIUS=0.2286  ASPECT_RATIO=0.45  MASS=11.2  IYY=1.084  br=0.01  GRAVITY=-9.81  zo=0  zdoto=0  BREFF=8.25094594147963  DREFF=0.260468730454265  FREFF=0.0735298544471851  Q_RE0=1.00866439868088  Q_V1=0.000760413786224011  Q_V2=0.0463384792019201  Q_FZ1=0  Q_FZ2=15.6870832810226  Q_FZ3=0  Q_FCX=0.138643970247602  Q_FCY=0.10843499565426  Q_FCY2=-0.465763352339538  PFZ1=0.69958166705601  VERTICAL_STIFFNESS=207885.061134007  VERTICAL_DAMPING=500  BOTTOM_OFFST=0.00990653336182505  BOTTOM_STIFF=1999075.87051971  Q_CAM1=86.7791723017291  Q_CAM2=259.705254231766  Q_CAM3=0.510281667378416  Q_FYS1=-20769.4728880343  Q_FYS2=-59060.183485617  Q_FYS3=89271.8260126986  LONGITUDINAL_STIFFNESS=388714.175879854  LATERAL_STIFFNESS=157087.404633332  PCFX1=0.18539229191199  PCFX2=0  PCFX3=0  PCFY1=0.163183345037677  PCFY2=0  PCFY3=0.249094918231954  Q_RA1=0.675942571700787  Q_RA2=0.73800463546164  Q_RB1=1.04487486456705  Q_RB2=-1.191763806629  PCX1=1.58523057950359  PDX1=1.7  PDX2=-0.0842405110022724  PDX3=0  PEX1=0.110312777158455  PEX2=0.313468516038146  PEX3=0  PEX4=0.0016060905760045  PKX1=21.3872544684023  PKX2=14.0006541873175  PKX3=-0.405326109653452  PHX1=0.000212599305364818  PHX2=0.00115950515263055  PVX1=1.59236164471432e-05  PVX2=0.000104321112127671  PPX1=-0.349461321276586  PPX2=0.387840040616429  PPX3=-0.0969947336569324  PPX4=0.0632271859795801  RBX1=12.7633329850276  RBX2=9.5787123658471  RBX3=0  RCX1=1.02796280922059  REX1=-0.45202516851367  REX2=-0.47304886171176  RHX1=0.000233272373115809  QSX1=-0.00788307788961443  QSX2=0.954629515459396  QSX3=0.0155855777667025  QSX4=0.125904607142414  QSX5=1.01110069703963  QSX6=20.1938577118433  QSX7=0.310818120717083  QSX8=-0.0430823751139655  QSX9=0.636494404888216  QSX10=0.142438060591663  QSX11=0.346766530036373  QSX12=0  QSX13=0  QSX14=0  PPMX1=0  PCY1=1.34299950037631  PDY1=0.878267729082195  PDY2=-0.0644597923147385  PDY3=0  PEY1=-0.809776534470972  PEY2=-0.600180598867198  PEY3=0.0991732552633487  PEY4=-6.5577974035573  PEY5=0  PKY1=-15.5714726518315  PKY2=1.73126522291751  PKY3=0.365349873517229  PKY4=1.98176755955416  PKY5=0  PKY6=-0.884005199550313  PKY7=-0.237259727611847  PHY1=-0.00183370557235628  PHY2=0.00346401302716671  PVY1=-0.00675427560163264  PVY2=0.036379218103843  PVY3=-0.163543984089166  PVY4=-0.491003349625726  PPY1=-0.62059646553185  PPY2=-0.0647824842338686  PPY3=-0.164648843290686  PPY4=0.283193909060098  PPY5=0  RBY1=10.7588809173639  RBY2=7.70420065295029  RBY3=3.40283755070691e-06  RBY4=0  RCY1=1.06691874059059  REY1=0.308244924574305  REY2=7.48775032604508e-06  RHY1=0.0118479204960415  RHY2=7.63650177161071e-06  RVY1=0.0560024425050078  RVY2=7.48487127056197e-06  RVY3=0  RVY4=98.4047026517149  RVY5=2.02759273900054  RVY6=15.7623064923347  QSY1=0.00699077564863536  QSY2=0  QSY3=0.00153535478298811  QSY4=8.55710322455322e-05  QSY5=0  QSY6=0  QSY7=0.89443879773793  QSY8=-0.403227641260894  QBZ1=11.666656027484  QBZ2=-1.30355438574485  QBZ3=0  QBZ4=0.177918305399071  QBZ5=-0.162481135068033  QBZ6=0  QBZ9=30.1445534682089  QBZ10=0  QCZ1=1.29026978207574  QDZ1=0.0886972644991399  QDZ2=-0.0058634820161856  QDZ3=0.3805597481383  QDZ4=0  QDZ6=0.00160914918118959  QDZ7=-0.00211036330862154  QDZ8=-0.13921904912557  QDZ9=0.00816585550028243  QDZ10=0  QDZ11=0  QEZ1=-2.19802254534746  QEZ2=1.01850535789165  QEZ3=0  QEZ4=0.278379679112054  QEZ5=-0.548414722765386  QHZ1=0.00148361198869669  QHZ2=0.00202017567585904  QHZ3=0.240316641332066  QHZ4=-0.210114035738085  PPZ1=-0.443927982388615  PPZ2=0  SSZ1=0.00914999585397887  SSZ2=0.0389830656052735  SSZ3=0  SSZ4=0  PDXP1=0.396718274678791  PDXP2=0  PDXP3=0  PKYP1=1.00587060633573  PDYP1=0.40483048923438  PDYP2=0  PDYP3=0  PDYP4=0  PHYP1=0.992731942067188  PHYP2=0.150352945499914  PHYP3=0  PHYP4=-3.98988682633674  PECP1=0.502379254513503  PECP2=0  QDTP1=10.0178654287947  QCRP1=0.200627747200702  QCRP2=0.0995735881599772  QBRP1=0.0997107127960717  QDRP1=1.01432910167423  QDRP2=0  aMode=2
  Constant{,1..3,6,18..27,29..30,32} (18 alike) : Constant  Value=0
  Constant{10..13} (4 alike) : Constant  Value=262000
  Constant{14..17} (4 alike) : Constant  Value=[1; 2.3; ones(25,1)]
  FxFL : Outport
  FxFR : Outport  Port=2
  FxRR : Outport  Port=3
  FxRL : Outport  Port=4
  tag scope: OmegaRL=global, OmegaRR=global
  wires:
  Constant12/1 -> Combined Slip Wheel 2DOF Front Right/7
  Constant16/1 -> Combined Slip Wheel 2DOF Front Right/10
  Constant26/1 -> Combined Slip Wheel 2DOF Rear Right/6
  Constant22/1 -> Combined Slip Wheel 2DOF Front Right/6
  Constant10/1 -> Combined Slip Wheel 2DOF Rear Left/7
  Combined Slip Wheel 2DOF Rear Right/3 -> FxRR/1
  [VxFR] -> Combined Slip Wheel 2DOF Front Right/3
  FzRR/1 -> Combined Slip Wheel 2DOF Rear Right/9
  Constant27/1 -> Combined Slip Wheel 2DOF Rear Right/8
  Constant18/1 -> Combined Slip Wheel 2DOF Front Left/5
  [BFL] -> Combined Slip Wheel 2DOF Front Left/1
  [VxFL] -> Combined Slip Wheel 2DOF Front Left/3
  [AxlTrqRR] -> Combined Slip Wheel 2DOF Rear Right/2
  Constant24/1 -> Combined Slip Wheel 2DOF Rear Left/6
  Constant30/1 -> Combined Slip Wheel 2DOF Rear Left/4
  Constant14/1 -> Combined Slip Wheel 2DOF Front Left/10
  Constant6/1 -> Combined Slip Wheel 2DOF Front Left/4
  Constant11/1 -> Combined Slip Wheel 2DOF Rear Right/7
  [VxRR] -> Combined Slip Wheel 2DOF Rear Right/3
  [BRR] -> Combined Slip Wheel 2DOF Rear Right/1
  Combined Slip Wheel 2DOF Rear Left/3 -> FxRL/1
  Constant1/1 -> Combined Slip Wheel 2DOF Rear Right/5
  Constant20/1 -> Combined Slip Wheel 2DOF Front Left/8
  Constant13/1 -> Combined Slip Wheel 2DOF Front Left/7
  [BRL] -> Combined Slip Wheel 2DOF Rear Left/1
  FzRL/1 -> Combined Slip Wheel 2DOF Rear Left/9
  [AxlTrqRL] -> Combined Slip Wheel 2DOF Rear Left/2
  Constant17/1 -> Combined Slip Wheel 2DOF Rear Right/10
  Constant23/1 -> Combined Slip Wheel 2DOF Front Right/8
  FzFR/1 -> Combined Slip Wheel 2DOF Front Right/9
  Constant32/1 -> Combined Slip Wheel 2DOF Rear Right/4
  Combined Slip Wheel 2DOF Front Left/3 -> FxFL/1
  Constant/1 -> Combined Slip Wheel 2DOF Rear Left/5
  Constant19/1 -> Combined Slip Wheel 2DOF Front Left/6
  Constant25/1 -> Combined Slip Wheel 2DOF Rear Left/8
  FzFL/1 -> Combined Slip Wheel 2DOF Front Left/9
  Combined Slip Wheel 2DOF Rear Left/2 -> [OmegaRL]
  Combined Slip Wheel 2DOF Rear Right/2 -> [OmegaRR]
  [VxRL] -> Combined Slip Wheel 2DOF Rear Left/3
  Constant15/1 -> Combined Slip Wheel 2DOF Rear Left/10
  [BFR] -> Combined Slip Wheel 2DOF Front Right/1
  Constant21/1 -> Combined Slip Wheel 2DOF Front Right/5
  Constant29/1 -> Combined Slip Wheel 2DOF Front Right/4
  Combined Slip Wheel 2DOF Front Right/3 -> FxFR/1
  Constant2/1 -> Combined Slip Wheel 2DOF Front Left/2
  Constant3/1 -> Combined Slip Wheel 2DOF Front Right/2
